simulink model "EINT_system_simulationPID"  (R2026b)
settings: Solver=FixedStepAuto  StopTime=50  FixedStep=0.05
values from neighbouring files (symbols this model uses):
  Ts = 0.05    [generate_db_ext.m]    (also in generate_db_mvt_z.m; generate_db_regime_z.m; generate_db_thrustrollyawpitch.m; plot_db_ext.m)
libraries: slpidlib x6
settings Model: Creator=Max  LastModifiedBy=hp

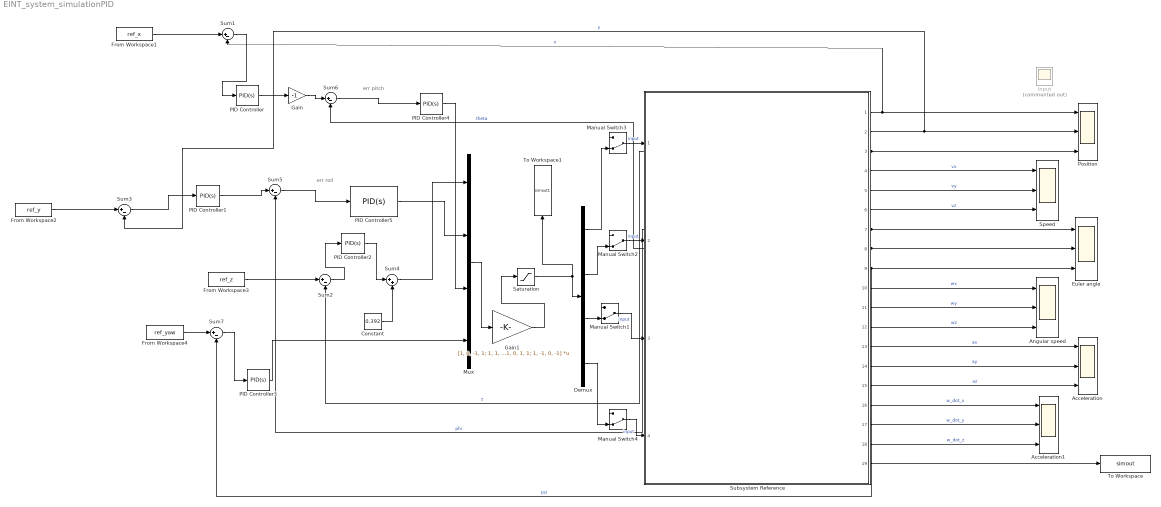
== system EINT_system_simulationPID ==
  note: err roll
  note: err pitch
  Acceleration : Scope  NumInputPorts=3
      settings: ActiveDisplayYMinimum=-35.281005723766839  ActiveDisplayYMaximum=15.731146517352213
  Acceleration1 : Scope  NumInputPorts=3
      settings: ActiveDisplayYMinimum=-0.001685836058753215  ActiveDisplayYMaximum=0.0017198230377338379  DataLoggingVariableName=ScopeData2
  Angular speed : Scope  NumInputPorts=3
      settings: ActiveDisplayYMinimum=-0.0017944152997961444  ActiveDisplayYMaximum=0.0013870133773098228  DataLoggingVariableName=ScopeData3
  Constant : Constant  Value=0.392
  Demux : Demux
  Euler angle : Scope  NumInputPorts=3
      settings: ActiveDisplayYMinimum=-0.0015056708614162  ActiveDisplayYMaximum=0.0014608574763041245  DataLoggingVariableName=ScopeData4
  From Workspace1 : FromWorkspace  VariableName=ref_x
  From Workspace2 : FromWorkspace  VariableName=ref_y
  From Workspace3 : FromWorkspace  VariableName=ref_z
  From Workspace4 : FromWorkspace  VariableName=ref_yaw
  Gain : Gain  Gain=-1
  Gain1 : Gain  Gain=[1, 0, -1, 1; 1, 1, 0, -1; 1, 0, 1, 1; 1, -1, 0, -1]  Multiplication=Matrix(K*u)
  Input : Scope  Commented=on
      settings: ActiveDisplayYMinimum=-1.25  ActiveDisplayYMaximum=1.25  DataLoggingVariableName=ScopeData5
  Manual Switch{1..4} (4 alike) : ManualSwitch  CurrentSetting=0
  Mux : Mux
  PID Controller{,1..5} (6 alike) : slpidlib/PID Controller  Controller=PID  Form=Parallel  TimeDomain=Continuous-time  UseExternalTs=off  SampleTime=-1  IntegratorMethod=Forward Euler  FilterMethod=Forward Euler  ControllerParametersSource=internal  P=0  I=0  UseKiTs=off  D=0  UseExternalDerivativeSource=off  N=100  UseFilter=on  TunerSelectOption=Transfer Function Based (PID Tuner App)  InitialConditionSource=internal  InitialConditionForIntegrator=0  InitialConditionForFilter=0  DifferentiatorICPrevScaledInput=0  ExternalReset=none  TrackingMode=off  Kt=1  LimitOutput=off  SatLimitsSource=internal  UpperSaturationLimit=inf  LowerSaturationLimit=-inf  LinearizeAsGain=on  AntiWindupMode=none  Kb=1  LimitIntegrator=off  UpperIntegratorSaturationLimit=inf  LowerIntegratorSaturationLimit=-inf  POutMin=[]  POutMax=[]  IOutMin=[]  IOutMax=[]  DOutMin=[]  DOutMax=[]  NOutMin=[]  NOutMax=[]  SumOutMin=[]  SumOutMax=[]  SaturationOutMin=[]  SaturationOutMax=[]  PParamMin=[]  PParamMax=[]  IParamMin=[]  IParamMax=[]  DParamMin=[]  DParamMax=[]  NParamMin=[]  NParamMax=[]  KbParamMin=[]  KbParamMax=[]  KtParamMin=[]  KtParamMax=[]  KbOutMin=[]  KbOutMax=[]  KtOutMin=[]  KtOutMax=[]  IntegratorOutMin=[]  IntegratorOutMax=[]  FilterOutMin=[]  FilterOutMax=[]  SumI1OutMin=[]  SumI1OutMax=[]  SumI2OutMin=[]  SumI2OutMax=[]  SumI3OutMin=[]  SumI3OutMax=[]  SumI4OutMin=[]  SumI4OutMax=[]  SumDOutMin=[]  SumDOutMax=[]  DifferentiatorOutMin=[]  DifferentiatorOutMax=[]  FilterDiffOutCoefMin=[]  FilterDiffOutCoefMax=[]  ReciprocalOutMin=[]  ReciprocalOutMax=[]  SumDenOutMin=[]  SumDenOutMax=[]  SumNumOutMin=[]  SumNumOutMax=[]  DivideOutMin=[]  DivideOutMax=[]  UdiffTsProdOutMin=[]  UdiffTsProdOutMax=[]  NTsProdOutMin=[]  NTsProdOutMax=[]  UintegralTsProdOutMin=[]  UintegralTsProdOutMax=[]  UngainTsProdOutMin=[]  UngainTsProdOutMax=[]  ClampingZeroOutDataTypeStr=Inherit: Inherit via back propagation  ClampingZeroOutMin=[]  ClampingZeroOutMax=[]  FilterDenConstantOutDataTypeStr=Inherit: Inherit via back propagation  FilterDenConstantOutMin=[]  FilterDenConstantOutMax=[]  PCopyOutDataTypeStr=Inherit: Inherit via back propagation  PCopyOutMin=[]  PCopyOutMax=[]  NCopyOutDataTypeStr=Inherit: Inherit via back propagation  NCopyOutMin=[]  NCopyOutMax=[]  IntegratorContinuousStateAttributes=''  IntegratorStateMustResolveToSignalObject=off  IntegratorRTWStateStorageClass=Auto  FilterContinuousStateAttributes=''  FilterStateMustResolveToSignalObject=off  FilterRTWStateStorageClass=Auto  ParallelPVariant=InternalParameters  IdealPVariant=Disabled  IVariant=InternalParameters  DVariant=InternalParameters  IntegratorVariant=Continuous  SatVariant=Disabled  AWVariant=Passthrough  PCopyVariant=Disabled  TRVariant=Disabled  FdbkBlocksVariant=Forward  IdealPFdbkVariant=Disabled  SatFdbkVariant=Disabled  DerivativeFilterVariant=ContFilter  NVariant=InternalParameters  NCopyVariant=Disabled  FilterICVariant=InternalICsFilter  IntegratorICVariant=InternalICs  ExternalResetVariant=Disabled  TRSumVariant=Passthrough  SumFdbkVariant=Disabled  SumVariant=Sum_PID  TsampFilterVariant=InternalTs  TsampNgainVariant=Passthrough  TsampIntegralVariant=Disabled_SignalSpec  ExternalSaturationOutDataTypeStr=Inherit: Same as second input  DerivativeSourceVariant=ErrorSignal  PreIntVariant=InternalPreInt
  Position : Scope  NumInputPorts=3
      settings: ActiveDisplayYMinimum=-0.0017156213360334711  ActiveDisplayYMaximum=0.0017146351630340326  DataLoggingVariableName=ScopeData6
  Saturation : Saturate  UpperLimit=3  LowerLimit=-3
  Speed : Scope  NumInputPorts=3
      settings: ActiveDisplayYMinimum=-0.0017455024957211969  ActiveDisplayYMaximum=0.0017346711746104369
  Subsystem Reference : Subsystem  ReferencedSubsystem=UAV_model
  Sum{1..3,5..7} (6 alike) : Sum  Inputs=|+-
  Sum4 : Sum  Inputs=|++
  To Workspace : ToWorkspace  VariableName=simout  SampleTime=Ts
  To Workspace1 : ToWorkspace  VariableName=simout1  SampleTime=-1
  wires:
  Subsystem Reference/18 -> Acceleration1/3  "w_dot_z"
  Subsystem Reference/12 -> Angular speed/3  "wz"
  Subsystem Reference/17 -> Acceleration1/2  "w_dot_y"
  Subsystem Reference/9 -> Sum7/2, Euler angle/3  "psi"
  Subsystem Reference/8 -> Euler angle/2, Sum6/2  "theta"
  Subsystem Reference/14 -> Acceleration/2  "ay"
  Subsystem Reference/10 -> Angular speed/1  "wx"
  Subsystem Reference/2 -> Sum3/2, Position/2  "y"
  Subsystem Reference/13 -> Acceleration/1  "ax"
  Subsystem Reference/15 -> Acceleration/3  "az"
  Subsystem Reference/16 -> Acceleration1/1  "w_dot_x"
  Subsystem Reference/7 -> Euler angle/1, Sum5/2  "phi"
  Subsystem Reference/19 -> To Workspace/1
  Subsystem Reference/1 -> Position/1, Sum1/2  "x"
  Subsystem Reference/6 -> Speed/3  "vz"
  Subsystem Reference/4 -> Speed/1  "vx"
  Subsystem Reference/3 -> Position/3, Sum2/2  "z"
  Subsystem Reference/5 -> Speed/2  "vy"
  Subsystem Reference/11 -> Angular speed/2  "wy"
  Manual Switch4/1 -> Subsystem Reference/4  "input"
  Manual Switch1/1 -> Subsystem Reference/3  "input"
  Manual Switch2/1 -> Subsystem Reference/2  "input"
  Manual Switch3/1 -> Subsystem Reference/1  "input"
  From Workspace1/1 -> Sum1/1
  From Workspace2/1 -> Sum3/1
  From Workspace3/1 -> Sum2/1
  Sum1/1 -> PID Controller/1
  Sum3/1 -> PID Controller1/1
  Sum2/1 -> PID Controller2/1
  PID Controller/1 -> Gain/1
  Constant/1 -> Sum4/2
  PID Controller1/1 -> Sum5/1
  Gain/1 -> Sum6/1
  Sum4/1 -> Mux/1
  From Workspace4/1 -> Sum7/1
  Mux/1 -> Gain1/1
  Gain1/1 -> Saturation/1
  Saturation/1 -> To Workspace1/1, Demux/1
  Demux/1 -> Manual Switch3/2
  Demux/2 -> Manual Switch2/2
  Demux/3 -> Manual Switch1/2
  Demux/4 -> Manual Switch4/2
  Sum7/1 -> PID Controller3/1
  PID Controller3/1 -> Mux/4
  PID Controller4/1 -> Mux/3
  Sum6/1 -> PID Controller4/1
  Sum5/1 -> PID Controller5/1
  PID Controller5/1 -> Mux/2
  PID Controller2/1 -> Sum4/1
